simulink model "Dll_Control_AFO_V8_5_R2019b"  (R2019b)
settings: Solver=ode2  StartTime=0.0  StopTime=10  FixedStep=Ts  RelTol=1e-3
InitFcn:
  | modelDir=fileparts(get_param(bdroot,'FileName'));addpath(modelDir);rootDir=fileparts(modelDir);if isfolder(rootDir),addpath(rootDir);end;fmuDir=fullfile(rootDir,'fmu');if isfolder(fmuDir),addpath(fmuDir);end;if evalin('base','exist(''Wf0'',''var'')'),assignin('base','Wfb',evalin('base','Wf0'));end;
values from neighbouring files (symbols this model uses):
  A80 = 0.10573    [RunCtrlSysModelSHT.m]
  b11 = B(1,1)*1    [RunCtrlSysModelSHT.m]
  b21 = B(2,1)*1    [RunCtrlSysModelSHT.m]
  d31 = D(3,1)    [RunCtrlSysModelSHT.m]
  d41 = D(4,1)    [RunCtrlSysModelSHT.m]
  ExternalSecondaryAirEnabled = 0    [RunCtrlSysModelSHT.m]
  InitAir = zeros(50,1)    [RunCtrlSysModelSHT.m]
  Mkg0 = 0    [RunCtrlSysModelSHT.m]
  MkpDirectCommand = Mkp0    (= 999.278795578)    [RunCtrlSysModelSHT.m]
  MkpMax = 1200    [RunCtrlSysModelSHT.m]
  Ng0 = 38000    [RunCtrlSysModelSHT.m]
  NgMax = Ng0*1.05    (= 39900)    [RunCtrlSysModelSHT.m]
  Np0 = 20800    [RunCtrlSysModelSHT.m]
  NpDem = Np0    (= 20800)    [RunCtrlSysModelSHT.m]
  omega_u = 20    [RunCtrlSysModelSHT.m]
  power0 = 2176600    [RunCtrlSysModelSHT.m]
  RotorLoadCfg = struct(      'designNpRpm', Np0,      'designPowerW', power0,      'thetaZeroDeg', 0,      'thetaDesignDeg', 12,      'profileTorqueFraction', 0.15,      'thetaValidRangeDeg', [6, 14])    [RunCtrlSysModelSHT.m]
  RotorLoadInputMode = 'legacyPower'    [RunCtrlSysModelSHT.m]
  T45Max = 1400    [RunCtrlSysModelSHT.m]
  ThetaCommandDeg = RotorLoadCfg.thetaDesignDeg    [RunCtrlSysModelSHT.m]
  Ts = 0.025    [RunCtrlSysModelSHT.m]
  Wf0 = 0.151914044493225    (= 0.151914044493)    [RunCtrlSysModelSHT.m]
  WfMax = Wf0*2    (= 0.303828088986)    [RunCtrlSysModelSHT.m]
  WfMin = Wf0*0.01    (= 0.00151914044493)    [RunCtrlSysModelSHT.m]
  WfRateLim = 1.5    [RunCtrlSysModelSHT.m]
undefined symbols (not defined in the file or in its folder): sigbuilder_block, Wfb
libraries: simulink x10
(part 4 of 4)

== matlab function Dll_Control_AFO_V8_5_R2019b/空气系统代理模型/G02_燃气涡轮一级出口/辨识等效面积/IdentifiedAreaLaw ==
  data: boundaryTP24 input; area output
function area = f(boundaryTP24)
%#codegen
indices = [1 2 3 4 5 6 7 8 17 18 19 20 23 24];
center = [1143.9851310850022 107995.87488112479 1622.2348189112549 1499845.6209487044 1622.2348189112549 1499845.6209487044 1622.2348189112549 1499845.6209487044 1383.1099749981283 803920.74791491474 701.05126049106082 1554244.1667862225 701.05126049106082 1554244.1667862225];
scale = [95.954376618145574 621.80388296676324 138.0910860203727 100531.17106538037 138.0910860203727 100531.17106538037 138.0910860203727 100531.17106538037 117.02019532436552 50576.000521072063 15.06449605558042 104177.37934236297 15.06449605558042 104177.37934236297];
beta = [-8.2075887448017149 0.15394191740038604 0.026900652967621078 -0.074156472478261348 -0.0042485390902463147 -0.074156472465753132 -0.0042485390902615196 -0.074156472465753118 -0.0042485390803160637 0.019360132289856481 -0.0040571073038026938 0.0046230994432607565 -0.0042485464216748233 0.0046230994449429725 -0.0042485405656283396];
features = zeros(1, 14);
for k = 1:14
    features(k) = (boundaryTP24(indices(k)) - center(k)) / scale(k);
end
logArea = beta(1);
for k = 1:14
    logArea = logArea + features(k) * beta(k + 1);
end
logArea = min(0, max(-30, logArea));
area = exp(logArea);
end

== matlab function Dll_Control_AFO_V8_5_R2019b/空气系统代理模型/G03_燃气涡轮二级进口/辨识等效面积/IdentifiedAreaLaw ==
  data: boundaryTP24 input; area output
function area = f(boundaryTP24)
%#codegen
indices = [1 2 3 4 5 6 7 8 17 18 19 20 23 24];
center = [1143.9851310850022 107995.87488112479 1622.2348189112549 1499845.6209487044 1622.2348189112549 1499845.6209487044 1622.2348189112549 1499845.6209487044 1383.1099749981283 803920.74791491474 701.05126049106082 1554244.1667862225 701.05126049106082 1554244.1667862225];
scale = [95.954376618145574 621.80388296676324 138.0910860203727 100531.17106538037 138.0910860203727 100531.17106538037 138.0910860203727 100531.17106538037 117.02019532436552 50576.000521072063 15.06449605558042 104177.37934236297 15.06449605558042 104177.37934236297];
beta = [-8.547123623730787 0.15410650548147845 0.026737865043864918 -0.074217632394825303 -0.0042227284357218954 -0.074217632377167164 -0.0042227284357112703 -0.07421763237716715 -0.0042227284179119431 0.019391526152776953 -0.0040324563213518889 0.0048255695132650121 -0.0042227369341137555 0.0048255695010225403 -0.0042227308115121874];
features = zeros(1, 14);
for k = 1:14
    features(k) = (boundaryTP24(indices(k)) - center(k)) / scale(k);
end
logArea = beta(1);
for k = 1:14
    logArea = logArea + features(k) * beta(k + 1);
end
logArea = min(0, max(-30, logArea));
area = exp(logArea);
end

== matlab function Dll_Control_AFO_V8_5_R2019b/空气系统代理模型/G04_燃气涡轮二级出口/辨识等效面积/IdentifiedAreaLaw ==
  data: boundaryTP24 input; area output
function area = f(boundaryTP24)
%#codegen
indices = [1 2 3 4 5 6 7 8 17 18 19 20 23 24];
center = [1143.9851310850022 107995.87488112479 1622.2348189112549 1499845.6209487044 1622.2348189112549 1499845.6209487044 1622.2348189112549 1499845.6209487044 1383.1099749981283 803920.74791491474 701.05126049106082 1554244.1667862225 701.05126049106082 1554244.1667862225];
scale = [95.954376618145574 621.80388296676324 138.0910860203727 100531.17106538037 138.0910860203727 100531.17106538037 138.0910860203727 100531.17106538037 117.02019532436552 50576.000521072063 15.06449605558042 104177.37934236297 15.06449605558042 104177.37934236297];
beta = [-9.0416658885781711 0.15470826845596988 0.026143625946479013 -0.074441313835194936 -0.0041283817757420743 -0.074441313814669022 -0.0041283817757481267 -0.07444131381466898 -0.0041283817673592174 0.019506263848337837 -0.0039423428852018239 0.0056466861591913742 -0.0041283916611437313 0.0056466861786025344 -0.004128385165112965];
features = zeros(1, 14);
for k = 1:14
    features(k) = (boundaryTP24(indices(k)) - center(k)) / scale(k);
end
logArea = beta(1);
for k = 1:14
    logArea = logArea + features(k) * beta(k + 1);
end
logArea = min(0, max(-30, logArea));
area = exp(logArea);
end

== matlab function Dll_Control_AFO_V8_5_R2019b/空气系统代理模型/G05_动力涡轮一级叶根进口/辨识等效面积/IdentifiedAreaLaw ==
  data: boundaryTP24 input; area output
function area = f(boundaryTP24)
%#codegen
indices = [9 10 13 14 15 16 17 18 21 22];
center = [865.43799674365937 107995.87488112479 1143.9851310850022 107995.87488112479 1004.7115639143307 107995.87488112479 1383.1099749981283 803920.74791491474 472.63588966354899 735995.25555236544];
scale = [70.62227949731033 621.80388296676324 95.954376618145574 621.80388296676324 83.19897935159905 621.80388296676324 117.02019532436552 50576.000521072063 6.9143103070211733 45629.692151955103];
beta = [-10.393572517817208 -0.021595200261011586 0.0016723011124907482 0.25633548335581258 0.0016723016966698643 0.13865199512291429 0.0016723016966698628 -0.42664559456926804 0.0055902015756587702 0.0016121127972101301 0.0056143839642077403];
features = zeros(1, 10);
for k = 1:10
    features(k) = (boundaryTP24(indices(k)) - center(k)) / scale(k);
end
logArea = beta(1);
for k = 1:10
    logArea = logArea + features(k) * beta(k + 1);
end
logArea = min(0, max(-30, logArea));
area = exp(logArea);
end

== matlab function Dll_Control_AFO_V8_5_R2019b/空气系统代理模型/G06_动力涡轮一级叶根出口/辨识等效面积/IdentifiedAreaLaw ==
  data: boundaryTP24 input; area output
function area = f(boundaryTP24)
%#codegen
indices = [9 10 13 14 15 16 17 18 21 22];
center = [865.43799674365937 107995.87488112479 1143.9851310850022 107995.87488112479 1004.7115639143307 107995.87488112479 1383.1099749981283 803920.74791491474 472.63588966354899 735995.25555236544];
scale = [70.62227949731033 621.80388296676324 95.954376618145574 621.80388296676324 83.19897935159905 621.80388296676324 117.02019532436552 50576.000521072063 6.9143103070211733 45629.692151955103];
beta = [-10.592522614191168 -0.021468893361666904 0.001591569671777738 0.25639412180345234 0.0015915702533596337 0.13873941674731821 0.0015915702533596315 -0.42692057524324178 0.0057602978168393463 0.001708346249102137 0.0057860302936650074];
features = zeros(1, 10);
for k = 1:10
    features(k) = (boundaryTP24(indices(k)) - center(k)) / scale(k);
end
logArea = beta(1);
for k = 1:10
    logArea = logArea + features(k) * beta(k + 1);
end
logArea = min(0, max(-30, logArea));
area = exp(logArea);
end

== matlab function Dll_Control_AFO_V8_5_R2019b/空气系统代理模型/G07_动力涡轮二级叶尖进口/辨识等效面积/IdentifiedAreaLaw ==
  data: boundaryTP24 input; area output
function area = f(boundaryTP24)
%#codegen
indices = [9 10 11 12 13 14 15 16 21 22];
center = [865.43799674365937 107995.87488112479 539.63673770094624 971860.60007173312 1143.9851310850022 107995.87488112479 1004.7115639143307 107995.87488112479 472.63588966354899 735995.25555236544];
scale = [70.62227949731033 621.80388296676324 9.3566188709448621 62506.42760541787 95.954376618145574 621.80388296676324 83.19897935159905 621.80388296676324 6.9143103070211733 45629.692151955103];
beta = [-10.465262652791443 -0.014226823252058672 0.01075482525012381 0.65231726867037232 -0.024050963448591346 -0.014850186216870918 0.010754825117612785 -0.014601569309890027 0.010754825205077864 -0.630338867298463 -0.024050968423210424];
features = zeros(1, 10);
for k = 1:10
    features(k) = (boundaryTP24(indices(k)) - center(k)) / scale(k);
end
logArea = beta(1);
for k = 1:10
    logArea = logArea + features(k) * beta(k + 1);
end
logArea = min(0, max(-30, logArea));
area = exp(logArea);
end

== matlab function Dll_Control_AFO_V8_5_R2019b/空气系统代理模型/G08_动力涡轮二级叶尖出口/辨识等效面积/IdentifiedAreaLaw ==
  data: boundaryTP24 input; area output
function area = f(boundaryTP24)
%#codegen
indices = [9 10 11 12 13 14 15 16 21 22];
center = [865.43799674365937 107995.87488112479 539.63673770094624 971860.60007173312 1143.9851310850022 107995.87488112479 1004.7115639143307 107995.87488112479 472.63588966354899 735995.25555236544];
scale = [70.62227949731033 621.80388296676324 9.3566188709448621 62506.42760541787 95.954376618145574 621.80388296676324 83.19897935159905 621.80388296676324 6.9143103070211733 45629.692151955103];
beta = [-10.733139080297843 -0.014243711061168944 0.010764221045966416 0.6522188855599742 -0.024069312343939463 -0.014835165561398281 0.01076422090882552 -0.014600075977760436 0.010764220994587603 -0.6302583156000916 -0.024069317948024988];
features = zeros(1, 10);
for k = 1:10
    features(k) = (boundaryTP24(indices(k)) - center(k)) / scale(k);
end
logArea = beta(1);
for k = 1:10
    logArea = logArea + features(k) * beta(k + 1);
end
logArea = min(0, max(-30, logArea));
area = exp(logArea);
end

== matlab function Dll_Control_AFO_V8_5_R2019b/滑油系统代理模型/AB轴承腔通风模块/四封严双腔通风计算 ==
  data: boundary10 input; cavityState8 output; speed2 input; leak4 output; vent3 output; sealDP4 output; ventDP2 output; residual2 output
function [cavityState8, leak4, vent3, sealDP4, ventDP2, residual2] = fcn(boundary10, speed2)
%#codegen
paf=max(boundary10(1),1000); taf=max(boundary10(2),200);
par=max(boundary10(3),1000); tar=max(boundary10(4),200);
pbf=max(boundary10(5),1000); tbf=max(boundary10(6),200);
pbr=max(boundary10(7),1000); tbr=max(boundary10(8),200);
pvent=max(boundary10(9),1000); ng=max(speed2(1),1);
[pa,waf,war,ta,wva]=solveChamber(paf,taf,par,tar,pvent,ng,2.8806128155084619e-05,0.00028320121852302093,-2.2146841146971394,0.44366585815100312,0.00056714869278324143);
[pb,wbf,wbr,tb,wvb]=solveChamber(pbf,tbf,pbr,tbr,pvent,ng,0.00037638273444529552,0.00012675456754067898,1.6793213315973823,2.014934595412182,0.00082412591355737763);
cavityState8=[pa;ta;pa;ta;pb;tb;pb;tb];
leak4=[waf;war;wbf;wbr]; vent3=[wva;wvb;wva+wvb];
sealDP4=[max(paf-pa,0);max(par-pa,0);max(pbf-pb,0);max(pbr-pb,0)];
ventDP2=[max(pa-pvent,0);max(pb-pvent,0)];
residual2=[waf+war-wva;wbf+wbr-wvb];
end

function [pc,w1,w2,tmix,wvent]=solveChamber(p1,t1,p2,t2,pvent,ng,k1,k2,n1,n2,kv)
lo=pvent+1; hi=max(lo+1,min(p1,p2)-1);
for idx=1:50
  pc=0.5*(lo+hi);
  [r,w1,w2,tmix,wvent]=balance(pc,p1,t1,p2,t2,pvent,ng,k1,k2,n1,n2,kv);
  if r>0, lo=pc; else, hi=pc; end
end
pc=0.5*(lo+hi);
[~,w1,w2,tmix,wvent]=balance(pc,p1,t1,p2,t2,pvent,ng,k1,k2,n1,n2,kv);
end

function [r,w1,w2,tmix,wvent]=balance(pc,p1,t1,p2,t2,pvent,ng,k1,k2,n1,n2,kv)
sn=max(ng/38000,0.2);
w1=k1*sn^n1*sqrt(max(p1-pc,0)/max(t1,200));
w2=k2*sn^n2*sqrt(max(p2-pc,0)/max(t2,200));
tmix=(w1*t1+w2*t2)/max(w1+w2,1e-12);
wvent=kv*sqrt(max(pc-pvent,0)/max(tmix,200));
r=w1+w2-wvent;
end

== matlab function Dll_Control_AFO_V8_5_R2019b/滑油系统代理模型/FCN_Input_Adapter_5to26 ==
  data: u5 input; u26 output
function u26 = fcn(u5)
%#codegen
% Inputs 1:5 preserve the oil interface; 6:15 are VentBoundary10.
u26 = zeros(26,1);
mode = u5(1); Wf = u5(2); TaIn = u5(3); TinOil = u5(4); TinCool = u5(5);
if TaIn > 180
    Tair = TaIn; TaC = Tair - 273.15;
else
    TaC = TaIn; Tair = TaC + 273.15;
end
if ~isfinite(TinOil), TinOil = 83; end
if ~isfinite(TinCool), TinCool = TinOil; end
Paf=u5(6); Taf=u5(7); Par=u5(8); Tar=u5(9);
Pbf=u5(10); Tbf=u5(11); Pbr=u5(12); Tbr=u5(13);
Pvent=u5(14); Tvent=u5(15);
ventOK = isfinite(Paf) && isfinite(Taf) && isfinite(Par) && isfinite(Tar) ...
    && isfinite(Pbf) && isfinite(Tbf) && isfinite(Pbr) && isfinite(Tbr) ...
    && isfinite(Pvent) && isfinite(Tvent) ...
    && Paf>1e5 && Par>1e5 && Pbf>1e5 && Pbr>1e5 ...
    && Pvent>3e4 && Taf>250 && Tar>250 && Tbf>250 && Tbr>250 && Tvent>180;
if ~ventOK
    Paf=3.08e5; Par=3.08e5; Pbf=3.20e5; Pbr=3.20e5;
    Taf=472; Tar=472; Tbf=523; Tbr=558;
    Pvent=1.01325e5; Tvent=288.15;
end
Ttank = 352.15; if TaC < 0, Ttank = 345.15; end
TwallA = clamp1(0.5*(Taf+Tar),250,700);
TwallB = clamp1(0.5*(Tbf+Tbr),250,700);
PsealA = clamp1(0.5*(Paf+Par),1e5,5e5);
PsealB = clamp1(0.5*(Pbf+Pbr),1e5,5e5);
u26(1)=mode; u26(2)=Wf; u26(3)=TaC; u26(4)=TinOil; u26(5)=TinCool;
u26(6)=9000; u26(7)=11800; u26(8)=clamp1(TinOil+273.15,300,500);
u26(9)=Ttank; u26(10)=clamp1(Tair,250,1100); u26(11)=clamp1(TinCool,20,180);
u26(12)=TwallA; u26(13)=TwallB; u26(14)=468; u26(15)=485; u26(16)=438;
u26(17)=1.50e5; u26(18)=PsealA; u26(19)=PsealB;
u26(20)=clamp1(Pvent,3e4,2e5); u26(21)=clamp1(Tvent,250,360);
u26(22)=8.0e5; u26(23)=6.0e5; u26(24)=4.0e5; u26(25)=0; u26(26)=0;
end

function y=clamp1(x,lo,hi)
y=min(max(x,lo),hi);
end

== matlab function Dll_Control_AFO_V8_5_R2019b/滑油系统代理模型/散热器模块/燃滑空滑特性 ==
  data: oilInlet2C input; fuel2 output; air2 output
function [fuel2,air2]=fcn(oilInlet2C)
%#codegen
fuelTin=min(max(oilInlet2C(1),120),160);
airTin=min(max(oilInlet2C(2),100),180);
fuelTout=lookup5(fuelTin,[120,130,140,150,160],[100,107,112,120,126]);
fuelQ=lookup5(fuelTin,[120,130,140,150,160],[9.5,11,13.5,15,16.5]);
airTout=lookup5(airTin,[100,120,140,160,180],[84,100,115,130,144]);
airQ=lookup5(airTin,[100,120,140,160,180],[6.5,8.5,10.5,12.5,15.5]);
fuel2=[fuelTout;fuelQ]; air2=[airTout;airQ];
end

function y=lookup5(x,bp,tbl)
y=tbl(1);
if x>=bp(5), y=tbl(5); return; end
for idx=1:4
  if x>=bp(idx) && x<=bp(idx+1)
    f=(x-bp(idx))/(bp(idx+1)-bp(idx));
    y=tbl(idx)+f*(tbl(idx+1)-tbl(idx)); return;
  end
end
end

== matlab function Dll_Control_AFO_V8_5_R2019b/滑油系统代理模型/滑油系统代理核心/支路_燃滑散热/FCN_FuelOil_FP_Coupling ==
  data: QA input; y output; QB input; QG input; Pman input; PA input; PB input
function y = fcn(QA,QB,QG,Pman,PA,PB)
%#codegen
% Visible scalar coupling from flow-pressure branch.
qOil=max(QA+QB+QG,1e-9);
qRef=15.9/60000; qN=clamp1(qOil/qRef,0.2,2.5);
flowFactor=sqrt(qN);
Pdown=max(PA,PB);
Pin=max(Pman,Pdown+2.0e4);
dp=clamp1(0.03*Pin*qN^2,2.0e3,0.05*Pin);
Pout=max(Pdown+1.0e4,Pin-dp);
y=[flowFactor;Pin;Pout];
end
function y=clamp1(x,lo,hi)
y=min(max(x,lo),hi);
end

== matlab function Dll_Control_AFO_V8_5_R2019b/滑油系统代理模型/滑油系统代理核心/支路_流量压力分配/核心流量压力计算/FCN_FP_Formula ==
  data: u input; y output
function y = fcn(u)
%#codegen
% [QA QB PA PB QG Pman Pret], SI units.
NH=max(u(1),0); NL=max(u(2),0); cmd=clamp1(u(3),0,1);
vA=clamp1(u(4),0,1); vB=clamp1(u(5),0,1);
vG1=clamp1(u(6),0,1); vG2=clamp1(u(7),0,1); vG3=clamp1(u(8),0,1);
Ttank=clamp1(u(9),250,450);
Preturn=max(u(17),7.0e4); PsealA=max(u(18),7.0e4);
PsealB=max(u(19),7.0e4); Pvent=max(u(20),7.0e4);
filterCmd=clamp1(u(23),0,1);
rho=clamp1(860*(1-7e-4*(Ttank-353.15)),740,920);
mu=clamp1(0.020*exp(-0.017*(Ttank-353.15)),0.004,0.08);
nEq=0.45*NH+0.55*NL; spd=clamp1(nEq/14390,0.2,2.8);
qTotLpm=clamp1(15.9*cmd,2.0,45.0);
wA=7.9; wB=5.9; wG=2.1;
wSum=wA+wB+wG;
QA=qTotLpm*wA/wSum/60000;
QB=qTotLpm*wB/wSum/60000;
QG=qTotLpm*wG/wSum/60000;
dpPump=1.2e6*cmd*spd^1.5;
dpFilt=(0.08e6+0.22e6*filterCmd)*spd;
dpVis=8e4*(mu/0.020)^0.4*((QA+QB)*60000)/15.9;
Pman=clamp1(Preturn+max(dpPump-dpFilt-dpVis,1e4),4.0e5,1.3e6);
PA=Preturn+2.2e6*QA^2+0.25*PsealA;
PB=Preturn+2.6e6*QB^2+0.25*PsealB;
Pret=max(Preturn+1.6e6*(QA+QB)^2,Pvent+8000);
y=[QA;QB;PA;PB;QG;Pman;Pret];
end
function y=clamp1(x,lo,hi)
y=min(max(x,lo),hi);
end

== matlab function Dll_Control_AFO_V8_5_R2019b/滑油系统代理模型/滑油系统代理核心/支路_流量压力分配/核心流量压力计算/FCN_FP_Predict ==
  data: u input; y output
function y = fcn(u)
%#codegen
% Embedded deterministic FP residual.
% Coefficients can be entered here later; no external MAT/code dependency.
y = zeros(7,1);
if u(1) < -1e300
    y(1) = u(1);
end
end

== matlab function Dll_Control_AFO_V8_5_R2019b/滑油系统代理模型/滑油系统代理核心/支路_空滑换热/FCN_AOH_Formula ==
  data: u input; y output; QretA input; QretB input; Pret input
function y = fcn(u,QretA,QretB,Pret)
%#codegen
% Scalar direct coupling from flow-pressure branch.
NH=max(u(1),0); NL=max(u(2),0); cmd=clamp1(u(3),0,1.4);
Ttank=clamp1(u(9),250,450); Tair=clamp1(u(10),250,1100);
Pvent=max(u(20),7.0e4);
qOil=max((QretA+QretB)/0.96,1e-9);
qRef=13.8/60000; qN=clamp1(qOil/qRef,0.2,2.5);
TaC=Tair-273.15;
nN=clamp1((0.45*NH+0.55*NL)/20900,0.6,1.5);
QkW=(9.8-0.113*(TaC-35))*nN^0.35*(0.82+0.22*cmd)*qN^0.22;
Qdot=1000*clamp1(QkW,1.5,15.0);
mu=clamp1(0.020*exp(-0.017*(Ttank-353.15)),0.004,0.08);
Pin=max(Pret,Pvent+12000);
dp=clamp1(18000*qN^2*(mu/0.020)^0.25,2000,min(8.0e4,0.25*Pin));
Pout=max(Pvent+10000,Pin-dp);
y=[Qdot;Pin;Pout];
end
function y=clamp1(x,lo,hi)
y=min(max(x,lo),hi);
end

== matlab function Dll_Control_AFO_V8_5_R2019b/滑油系统代理模型/滑油系统代理核心/支路_空滑换热/FCN_AOH_Predict ==
  data: u input; y output
function y = fcn(u)
%#codegen
% Embedded deterministic AOH residual.
% Coefficients can be entered here later; no external MAT/code dependency.
y = zeros(3,1);
if u(1) < -1e300
    y(1) = u(1);
end
end

== matlab function Dll_Control_AFO_V8_5_R2019b/滑油系统代理模型/滑油系统代理核心/支路_轴承甲乙换热/FCN_BRG_Formula ==
  data: u input; y output
function y = fcn(u)
%#codegen
NH=max(u(1),0); NL=max(u(2),0); cmd=clamp1(u(3),0,1);
vA=clamp1(u(4),0,1); vB=clamp1(u(5),0,1);
vG=clamp1((u(6)+u(7)+u(8))/3,0,1);
Ttank=clamp1(u(9),250,450);
TwallA=clamp1(u(12),250,1100); TwallB=clamp1(u(13),250,1100);
PsealA=max(u(18),7e4); PsealB=max(u(19),7e4);
rho=clamp1(860*(1-7e-4*(Ttank-353.15)),740,920);
nEq=0.45*NH+0.55*NL; spd=clamp1(nEq/14390,0.2,2.8);
qTot=clamp1(15.9*cmd,2,45);
wA=7.9; wB=5.9; wS=wA+wB+2.1;
QA=qTot*wA/wS/60000; QB=qTot*wB/wS/60000;
nN=clamp1(nEq/20900,0.35,2.2); qs=nN^1.65;
QgenA=2811*qs*(0.92+0.12*cmd);
QgenB=4228*qs*(0.90+0.15*cmd);
mdA=max(QA*rho,0.03); mdB=max(QB*rho,0.03);
hA=420*(mdA/0.12)^0.72*(1+0.15*clamp1((PsealA-1.5e5)/2e5,0,1.5));
hB=420*(mdB/0.10)^0.72*(1+0.15*clamp1((PsealB-1.5e5)/2e5,0,1.5));
QdotA=clamp1(QgenA-hA*0.16*max(Ttank-TwallA,-40),-2e4,3e4);
QdotB=clamp1(QgenB-hB*0.16*max(Ttank-TwallB,-40),-2e4,3e4);
oilMass=max(u(22),0.4);
ToutA=clamp1(Ttank+QdotA/max(2000*(mdA+0.15*oilMass),500),260,520);
ToutB=clamp1(Ttank+QdotB/max(2000*(mdB+0.15*oilMass),500),260,520);
% Max-state AMESim calibration for bearing return-oil temperature.
% Targets: A=78.836 degC, B=78.195 degC.
ToutA=min(ToutA,351.986);
ToutB=min(ToutB,351.345);
y=[QdotA;QdotB;ToutA;ToutB];
end
function y=clamp1(x,lo,hi)
y=min(max(x,lo),hi);
end

== matlab function Dll_Control_AFO_V8_5_R2019b/滑油系统代理模型/滑油系统代理核心/支路_轴承甲乙换热/FCN_BRG_Predict ==
  data: u input; y output
function y = fcn(u)
%#codegen
% Embedded deterministic BRG residual.
% Coefficients can be entered here later; no external MAT/code dependency.
y = zeros(4,1);
if u(1) < -1e300
    y(1) = u(1);
end
end

== matlab function Dll_Control_AFO_V8_5_R2019b/滑油系统代理模型/滑油系统代理核心/支路机匣附件换热/FCN_CAS_Formula ==
  data: u input; y output
function y = fcn(u)
%#codegen
NH=max(u(1),0); NL=max(u(2),0); cmd=clamp1(u(3),0,1.4);
v=clamp1((u(6)+u(7)+u(8))/3,0,1);
Ttank=clamp1(u(9),250,450);
dT=(u(14)+u(15)+u(16))/3-Ttank;
nEq=0.45*NH+0.55*NL; nN=clamp1(nEq/20900,0.6,1.8);
spd=clamp1(nEq/14390,0.2,2.8);
qTot=clamp1(15.9*min(cmd,1),2,45);
wG=2.1; wS=7.9+5.9+wG;
QG=qTot*wG/wS/60000;
Qsrc=1800*nN^1.2*(0.70+0.50*cmd);
flowFactor=clamp1(QG/2.5e-4,0.4,2.2);
sepFactor=0.8+0.4*clamp1(u(24),0,1);
Qconv=260*(0.65+0.55*v)*flowFactor*sepFactor*dT;
y=clamp1(Qsrc+Qconv,0,2.5e4);
end
function y=clamp1(x,lo,hi)
y=min(max(x,lo),hi);
end

== matlab function Dll_Control_AFO_V8_5_R2019b/Turboshaft Engine Control System/Anti Integration Wind-Up ==
  data: dU_Schd input; dU output; Udelayed input; u_aLim input; u_dLim input; u_vLim input
function dU = fcn(dU_Schd, Udelayed, u_aLim, u_dLim, u_vLim)

Ts = 0.025;      %  u_vLim = 20;
if dU_Schd >  u_vLim*Ts
    dU_Schd = u_vLim*Ts;
elseif dU_Schd <  -u_vLim*Ts
    dU_Schd =  -u_vLim*Ts;
end

    if Udelayed >=  u_aLim
        if dU_Schd > 0
            dU_Schd = 0;
        end
    elseif Udelayed <= u_dLim
        if dU_Schd < 0
            dU_Schd = 0;
        end
    end
    
    if (Udelayed+dU_Schd) > u_aLim
        dU_Schd = u_aLim - Udelayed;
    elseif (Udelayed+dU_Schd) < u_dLim
        dU_Schd = u_dLim - Udelayed;
    end
    
dU = dU_Schd;

== matlab function Dll_Control_AFO_V8_5_R2019b/滑油系统代理模型/滑油系统代理核心/支路机匣附件换热/FCN_CAS_Predict ==
  data: u input; y output
function y = fcn(u)
%#codegen
% Embedded deterministic CAS residual.
% Coefficients can be entered here later; no external MAT/code dependency.
y = zeros(1,1);
if u(1) < -1e300
    y(1) = u(1);
end
end

== matlab function Dll_Control_AFO_V8_5_R2019b/FCN_G04_to_OilBoundaries ==
  data: g04T_K input; airTempC output; g04P_Pa input; ambientT_K input; ambientP_Pa input; ventBoundary10 output
function [airTempC, ventBoundary10] = fcn(g04T_K, g04P_Pa, ambientT_K, ambientP_Pa)
%#codegen
airTempC = 0;
ventBoundary10 = zeros(10,1);
[airTempC, ventBoundary10] = g04_to_oil_boundaries_fcn( ...
    g04T_K, g04P_Pa, ambientT_K, ambientP_Pa);
end

== matlab function Dll_Control_AFO_V8_5_R2019b/滑油系统代理模型/FCN_回油混合温度 ==
  data: tempA_C input; oilInlet2C output; tempB_C input; returnFlowA input; returnFlowB input
function oilInlet2C = fcn(tempA_C,tempB_C,returnFlowA,returnFlowB)
%#codegen
oilInlet2C = zeros(2,1);
oilInlet2C = oil_cooler_inlet_from_bearings_fcn( ...
    tempA_C,tempB_C,returnFlowA,returnFlowB);
end
